simulink model "Simulador"  (R2023b)
settings: Solver=VariableStepAuto  StartTime=0.0  StopTime=inf  RelTol=1e-3
undefined symbols (not defined in the file): f
libraries: instrumentlib x1
settings Model: Creator=oscarguerra  LastModifiedBy=oscarguerra

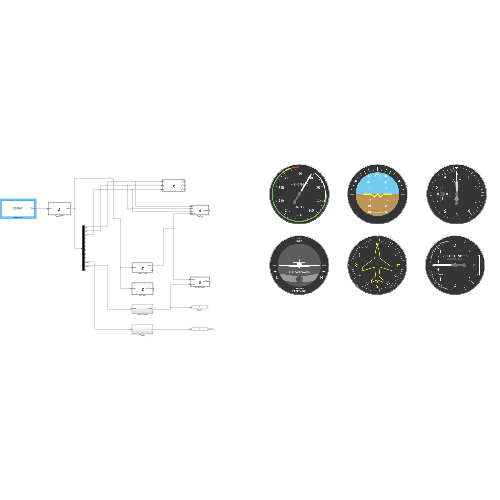
[thumbnail: Simulink's stored preview of the top-level diagram]
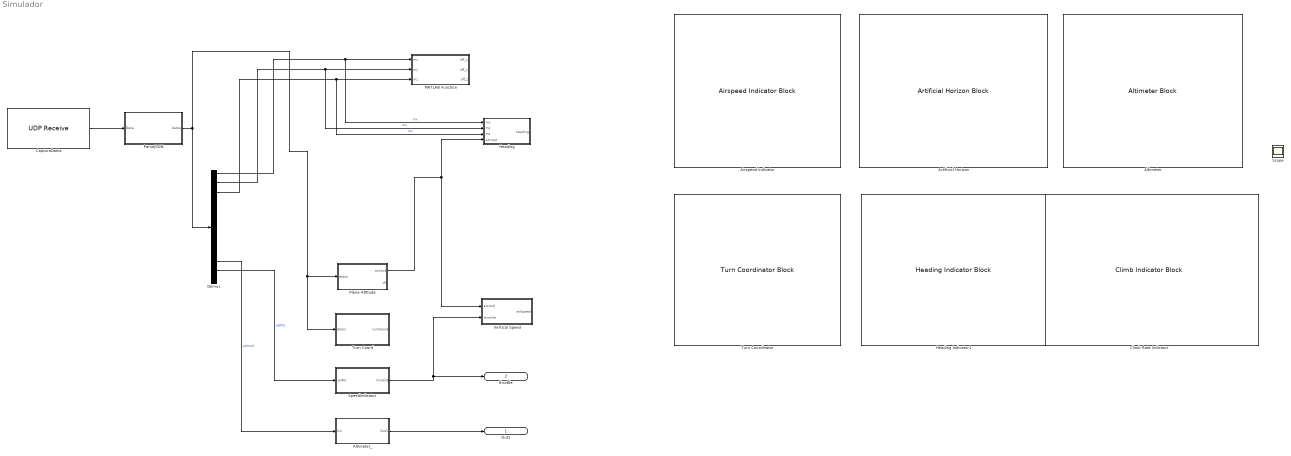
== system Simulador ==
  Airspeed Indicator : AirspeedIndicatorBlock  LabelPosition=Hide
  Altimeter : AltimeterBlock  LabelPosition=Hide
  Altimeter_ : Subsystem
  Artificial Horizon : ArtificialHorizonBlock  LabelPosition=Hide
  CapturaDatos : instrumentlib/UDP Receive  LocalAddress=192.168.1.34  LocalPort=65000  EnablePortSharing=off  Host=192.168.1.34  Port=65000  GetLatestData=off  DataSize=[1, 48]  DataType=uint8  ASCIIFormatting=%f,  Terminator=LF  CustomTerminator=10  ByteOrder=big-endian  EnableBlockingMode=on  Timeout=10  SampleTime=0.01  SimulateUsing=Interpreted execution
  Climb Rate Indicator : ClimbIndicatorBlock  LabelPosition=Hide
  Demux : Demux  Outputs=12
  Heading : MATLAB Function  TreatAsAtomicUnit=on
  Heading Indicator1 : HeadingIndicatorBlock  LabelPosition=Hide
  MATLAB Function : MATLAB Function  TreatAsAtomicUnit=on
  ParseJSON : MATLAB Function  TreatAsAtomicUnit=on
  Plane Attitude : MATLAB Function  TreatAsAtomicUnit=on
  SpeedIndicator : Subsystem
  Turn Coord : MATLAB Function  TreatAsAtomicUnit=on
  Turn Coordinator : TurnCoordinatorBlock  LabelPosition=Hide
  Vertical Speed : MATLAB Function  TreatAsAtomicUnit=on
  Out1 : Outport  SignalName=altitude
  throttle : Outport  Port=2
  Scope : Scope
  wires:
  CapturaDatos/1 -> ParseJSON/1(Data)
  Plane Attitude/1(actitud) -> Vertical Speed/1(actitud), Heading/4(actitud)
  ParseJSON/1(datos) -> Plane Attitude/1(datos), Turn Coord/1(datos), Demux/1
  Demux/10 -> Altimeter_/1(In1)  "altitud"
  Demux/11 -> SpeedIndicator/1(valPot)  "valPot"
  SpeedIndicator/1(throttle) -> Vertical Speed/2(throttle), throttle/1
  Altimeter_/1(Out1) -> Out1/1
  Demux/1 -> Heading/1(mx), MATLAB Function/1(mx)  "mx"
  Demux/2 -> Heading/2(my), MATLAB Function/2(my)  "my"
  Demux/3 -> Heading/3(mz), MATLAB Function/3(mz)  "mz"

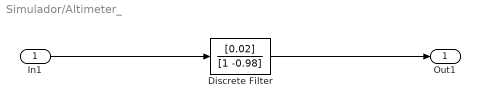
== system Simulador/Altimeter_ ==
  In1 : Inport
  Discrete Filter : DiscreteFilter  Numerator=[0.02]  Denominator=[1 -0.98]
  Out1 : Outport
  wires:
  In1/1 -> Discrete Filter/1
  Discrete Filter/1 -> Out1/1

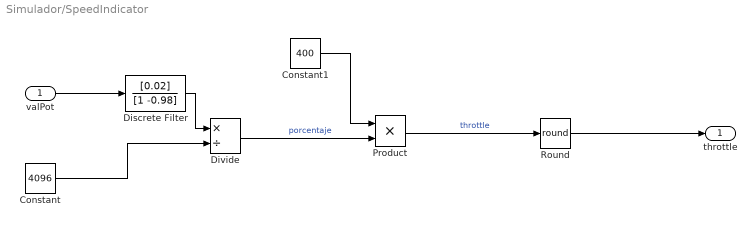
== system Simulador/SpeedIndicator ==
  valPot : Inport
  Constant : Constant  Value=4096
  Constant1 : Constant  Value=400
  Discrete Filter : DiscreteFilter  Numerator=[0.02]  Denominator=[1 -0.98]
  Divide : Product  Inputs=*/
  Product : Product
  Round : Rounding  Operator=round
  throttle : Outport
  wires:
  Constant/1 -> Divide/2
  Divide/1 -> Product/2  "porcentaje"
  Constant1/1 -> Product/1
  Round/1 -> throttle/1
  Product/1 -> Round/1  "throttle"
  valPot/1 -> Discrete Filter/1
  Discrete Filter/1 -> Divide/1

== matlab function Simulador/Heading ==
  data: mx input; my input; mz input; heading output; actitud input
function heading = fcn(mx, my, mz, actitud)
% Parámetros:
%   datos: Vector con datos de la IMU.
% Salida:
%   heading: Ma

    persistent headingPrev;

    roll = actitud(1);
    pitch = actitud(2);

    alpha = 0.05;
    mx_c = mx - (-1359.5);
    my_c = my - (-20.5);
    mz_c = mz - (2887.5);
    
    r = deg2rad(roll);
    p = deg2rad(pitch);

    Xh = mx_c * cos(p) + my_c * sin(r) * sin(p) + mz_c * cos(r) * sin(p);
    Yh = my_c * cos(r) - mz_c * sin(r);

    headingActual = rad2deg(atan2(-Yh, Xh));
    if (headingActual < 0), headingActual = headingActual + 360; end
    
    if isempty(headingPrev)
        headingPrev = headingActual;
    end

    diff = headingActual - headingPrev;
    if (diff > 180)
        diff = diff - 360;
    elseif (diff < -180)
        diff = diff + 360;
    end

    headingPrev = headingPrev + (alpha * diff);
    heading = mod(headingPrev, 360);
end

== matlab function Simulador/ParseJSON ==
  data: Data input; datos output
function datos = fcn(Data)
    datos = zeros(1,12, 'single');
    datos(1) = typecast(Data(1:4), 'single');               %% Mx.
    datos(2) = typecast(Data(5:8), 'single');               %% My.
    datos(3) = typecast(Data(9:12), 'single');              %% Mz.
    datos(4) = typecast(Data(13:16), 'single');             %% Ax.
    datos(5) = typecast(Data(17:20), 'single');             %% Ay.
    datos(6) = typecast(Data(21:24), 'single');             %% Az.
    datos(7) = typecast(Data(25:28), 'single');             %% Gx.
    datos(8) = typecast(Data(29:32), 'single');             %% Gy.
    datos(9) = typecast(Data(33:36), 'single');             %% Gz.
    datos(10) = typecast(Data(37:40), 'single');            %% Altitud
    datos(11) = typecast(Data(41:44), 'single');            %% Valor Potenciómetro.
    datos(12) = typecast(Data(45:48), 'single');            %% Tiempo Paquete.
end

== matlab function Simulador/MATLAB Function ==
  data: mx input; off_x output; my input; mz input; off_y output; off_z output
function [off_x, off_y, off_z] = fcn(mx, my, mz)
    % Variables que guardan su valor entre una llamada y otra
    persistent max_x min_x max_y min_y max_z min_z
    
    % Inicialización en la primera ejecución
    if isempty(max_x)
        max_x = mx; min_x = mx;
        max_y = my; min_y = my;
        max_z = mz; min_z = mz;
    end

    % Actualizar límites si el valor actual es mayor o menor
    if mx > max_x, max_x = mx; end
    if mx < min_x, min_x = mx; end
    
    if my > max_y, max_y = my; end
    if my < min_y, min_y = my; end
    
    if mz > max_z, max_z = mz; end
    if mz < min_z, min_z = mz; end

    % Calcular los offsets (Hard-Iron)
    off_x = (max_x + min_x) / 2;
    off_y = (max_y + min_y) / 2;
    off_z = (max_z + min_z) / 2;

    %disp(off_x);
    %disp(off_y);
    %disp(off_z);

end

== matlab function Simulador/Plane Attitude ==
  data: actitud output; datos input; dt output
function [actitud, dt]= fcn(datos)
% Parámetros:
%   datos: Vector con datos de la IMU.
% Salida:
%   actitud: Vector con roll y pitch (en º).

    ax = datos(4);
    ay = datos(5);
    az = datos(6);
    % Convertimos a radianes.
    gx = datos(7) * pi / 180;
    gy = datos(8) * pi / 180;
    gz = datos(9) * pi / 180;

    tiempoPaquete = datos(12) / 1000;

    alpha = 0.98;

    % Cálculos con acelerómetro.
    accRoll = atan2(-ay, -az);
    accPitch = atan2(ax, sqrt(ay^2 + az^2));

    % Cálculos con el giroscopio.
    persistent gyroRoll gyroPitch dtPrevio;
    if (isempty(gyroRoll) || isempty(gyroPitch))
        gyroRoll = accRoll;
        gyroPitch = accPitch;
        dtPrevio = tiempoPaquete;
       
    end
    dt = tiempoPaquete - dtPrevio;
    gyroRoll = gyroRoll + gx * dt;
    gyroPitch = gyroPitch + gy * dt;

    % Aplicamos Filtro Complementario.
    roll = alpha * gyroRoll + (1 - alpha) * accRoll;
    pitch = alpha * gyroPitch + (1 - alpha) * accPitch;

    % Guardamos los estados.
    dtPrevio = tiempoPaquete;
    gyroRoll = roll;
    gyroPitch = pitch;

    roll = roll * 180/pi;
    pitch = pitch * 180/pi;

    actitud = [roll; pitch];
end

== matlab function Simulador/Vertical Speed ==
  data: actitud input; throttle input; verSpeed output
function verSpeed = fcn(actitud, throttle)
% Parámetros:
%   throttle: Velocidad del avión en nudos.
%   actitud : Actitud/orientación del avión.
% Salida:
%   verSpeed: Velocidad vertical del avión en feets/min.



    throttle = double(throttle);
    pitch = double(actitud(2));

    maxVI = 4000;
    k = 101;

    persistent verSpeedFiltrada

    if isempty(verSpeedFiltrada)
        verSpeedFiltrada = 0.0;
    end

    % ----- Cálculo de velocidad vertical objetivo -----

    if throttle < 200

        % Descenso forzado
        verSpeedObjetivo = -1000.0;

    else

        if pitch > 5

            % Se empieza a contar el pitch a partir de 5º
            pitchEfectivo = pitch - 5;

            verSpeedObjetivo = throttle * k * sind(pitchEfectivo);

        elseif pitch < -5

            % Se empieza a contar el pitch a partir de -5º
            pitchEfectivo = pitch + 5;

            verSpeedObjetivo = throttle * k * sind(pitchEfectivo);

        else

            % Vuelo nivelado
            verSpeedObjetivo = 0.0;

        end
    end

    % Limitar a ±4000 ft/min
    verSpeedObjetivo = max(min(verSpeedObjetivo, maxVI), -maxVI);

    % ----- Suavizado exponencial -----

    alpha = 0.08;

    verSpeedFiltrada = verSpeedFiltrada + ...
        alpha * (verSpeedObjetivo - verSpeedFiltrada);

    % Salida
    verSpeed = single(verSpeedFiltrada);







    %maxVI = 4000;                   % Velocidad vertical máxima.
    
    %pitch = actitud(2);             % En grados º.

    %k = 101;

    %verSpeed_teorica = throttle * k * sind(pitch);

    %verSpeed = max(min(verSpeed_teorica, maxVI), -maxVI);

    %if (abs(verSpeed) < 50)
     %   verSpeed = single(0);
    %end

    %verSpeed = single(verSpeed);
    
    %if (throttle < 200)
        % Régimen de descenso.
    %    verSpeed = maxVI * sind(pitch);
    %else
    %    if (pitch > 5)
    %        % Régimen de ascenso.
    %        verSpeed = maxVI * sind(pitch);
    %    elseif ((pitch >= 0) && (pitch <= 5))
    %        % Vuelo nivelado.
    %        verSpeed = single(0);
    %    else
    %        % Régimen de descenso.
    %        verSpeed = maxVI * sind(pitch);
    %    end
    %end
end

== matlab function Simulador/Turn Coord ==
  data: datos input; turnCoord output
function turnCoord = fcn(datos)

    %% DATOS DE LA IMU
    Ay = double(datos(5));
    Az = double(datos(6));

    Gx = double(datos(7));
    Gz = double(datos(9));

    %% VARIABLES PERSISTENTES
    persistent biasGx biasGz biasAy signoZ
    persistent rateFiltrado bolaFiltrada
    persistent contador sumaGx sumaGz sumaAy sumaAz

    if isempty(contador)

        contador = 0;

        sumaGx = 0;
        sumaGz = 0;
        sumaAy = 0;
        sumaAz = 0;

        biasGx = 0;
        biasGz = 0;
        biasAy = 0;

        signoZ = 1;

        rateFiltrado = 0;
        bolaFiltrada = 0;
    end


    %% ---------------------------------------------------------
    % CALIBRACIÓN INICIAL
    % Mantener la IMU horizontal y quieta
    %% ---------------------------------------------------------

    if contador < 100

        contador = contador + 1;

        sumaGx = sumaGx + Gx;
        sumaGz = sumaGz + Gz;
        sumaAy = sumaAy + Ay;
        sumaAz = sumaAz + Az;

        biasGx = sumaGx / contador;
        biasGz = sumaGz / contador;
        biasAy = sumaAy / contador;

        if contador == 100

            if (sumaAz / contador) < 0
                signoZ = -1;
            else
                signoZ = 1;
            end

        end

        turnCoord = [0 0];
        return;
    end


    %% ---------------------------------------------------------
    % PARTE SUPERIOR DEL TURN COORDINATOR
    %% ---------------------------------------------------------

    % Eliminar bias del giroscopio
    gx = Gx - biasGx;
    gz = Gz - biasGz;

    % Zona muerta
    if abs(gx) < 0.5
        gx = 0;
    end

    if abs(gz) < 0.5
        gz = 0;
    end

    % Aproximación al giróscopo inclinado del TC
    rateTC = gz + gx * tand(30);

    % Suavizado
    alphaRate = 0.15;

    rateFiltrado = ...
        rateFiltrado + alphaRate * (rateTC - rateFiltrado);

    % Escalado para el instrumento
    turnIndicator = 5 * rateFiltrado;

    % Limitar a +-20 grados
    turnIndicator = ...
        max(min(turnIndicator,20),-20);


    %% ---------------------------------------------------------
    % BOLA DEL INCLINÓMETRO
    %% ---------------------------------------------------------

    % Eliminar offset lateral del acelerómetro
    ay = Ay - biasAy;

    % Asegurar componente vertical positiva
    azVertical = signoZ * Az;

    % Ángulo correspondiente a la aceleración lateral
    bola = atan2(ay,azVertical) * 180/pi;

    % Zona muerta
    if abs(bola) < 0.5
        bola = 0;
    end

    % Suavizado
    alphaBola = 0.10;

    bolaFiltrada = ...
        bolaFiltrada + alphaBola * (bola - bolaFiltrada);

    % Limitar a +-15 grados
    inclinometer = ...
        max(min(bolaFiltrada,15),-15);


    %% SALIDA
    turnCoord = [turnIndicator inclinometer];

end





%function turnCoord = fcn(datos, actitud)

 %   Gz = datos(9);
  %  roll = actitud(1);

   % turnRate = Gz/3;

    % 30° de alabeo -> bola al máximo
    %inclinometer = roll * 15/30;

    %inclinometer = max(min(inclinometer,15),-15);

%    turnCoord = [turnRate inclinometer];

%end
